simulink model "commhdlQPSKTxRxLoopback"  (R2025b)
settings: Solver=FixedStepDiscrete  StartTime=0.0  StopTime=0.03  RelTol=1e-3
PostLoadFcn:
  | hScopeConfig = get_param([gcs '/Receiver/QPSK Rx/Frequency and Time Synchronizer/Symbol Synchronizer/No HDL/QPSK Receiver Eye Diagram'],'ScopeConfiguration');
  | 
  | hScopeConfig.OpenAtSimulationStart = false;
  | hScopeConfig.Visible = false;
  | SamplesPerSymbol = 4;
  | %UpsamplesRx = 1;
  | clear hScopeConfig
InitFcn:
  | % RxAlign decoder latency (flat_simfix): 41 = netlist value used for HDL; set
  | % rxAlignLat = 25 in the base workspace before a model-level simulation.
  | if ~exist('rxAlignLat','var'), rxAlignLat = uint16(41); end
  | commhdlQPSKTxRxModelInit;
  | % Rate bridge: ADRV9002/Jupiter radio runs at 15.36 MHz = 2x the 7.68 MHz
  | % (4 samples/symbol @ Rsym=1.92 MHz) the QPSK Rx requires. The deployed
  | % Receiver must downsample the ADC stream by 2. UpsamplesRx=1 fed the QPSK
  | % Rx 8 sps (2x-upsampled) and broke symbol sync / the loopback bit check.
  | UpsamplesRx = 1;   %% T8 RATE FIX: rail 15.36e6 == ADC bus rate,
  | %% no ingress decimation (was 2 when the rail sat on the 7.68e6 rung)
  | UpsamplesTx = 1;
  | clear simTimingOffset;
StopFcn:
  | if exist('simTimingOffset','var')
  |   disp('Simulation completed');
  |   %QPSKTxRxVerification;
  | end
undefined symbols (not defined in the file or in its folder): Add, Config, fsym, randsrc, RandStream, Rsym, rxAlignLat, Shift
libraries: hdlsllib x141, simulink x45, dspsigops x30, dsphdlfiltering2 x6, dsphdlsigops2 x4, dsphdlmathfun2 x4, commdigbbndpm3 x4, dspmlti4 x2, commchan3 x1, commrflib2 x1, commcnvcod2 x1
(part 8 of 9)

== matlab function commhdlQPSKTxRxLoopback/TxRxComposite/Transmitter/Input Data/Message Generator/MATLAB Function ==
  data: enable input; reset input; out output; start output; stop output; valid output; count_out output; msg_count_out output
function [out, start, stop, valid, count_out, msg_count_out] = msggen(enable, reset)

persistent indexCount;
persistent toggle;
persistent msgCount;
persistent msgCountAll;
persistent msgCountBitIndex;

if isempty(indexCount) || isempty(toggle) || isempty(msgCount) || isempty(msgCountBitIndex) || isempty(msgCountAll)
    indexCount = uint32(0);
    msgCount = uint32(1);
    msgCountAll = uint32(1);
    msgCountBitIndex = uint8(0);
    toggle = false;
end

%% Constants -- FIXED pre-coded K=5 packet ROM (rom_words_1538_f3072.txt, 49216 bits,
%% word w = bits[32w..32w+31] MSB-first). Stored as 1538 x uint32 packed words
%% (a large inline logical literal crashes the Stateflow compiler),
%% unpacked into the 49216-element msgbits logical ROM and indexed with the
%% STOCK msgbits(indexCount+1) pattern. Replaces the stock 120-bit message ROM.
%% Content: K=5 [35 23] rate-1/2 coded info(24580)+tail(4) -> 49168 bits,
%% 3073x16 block-interleaved (perm r*16+c), + 48-bit PN9 filler. The K=5 Rx
%% deint(perm c*3073+r) + Viterbi(TB=25) recovers the 120-bit BIST message.
romWords = uint32([1204802801 1209539668 1975942268 2963809026 2596904318 4188557104 3596431864 4239974639 3463738471 2217388750 3654439215 3125256117 3023293192 2833794923 816778833 3181876726 1463245004 1536297995 531210280 521390638 503270692 25790812 3006566584 640748580 1552853862 3369715589 690379693 619729467 1586250071 2534918951 747314766 1864725699 736916321 2528559012 1966427766 2678711027 694905996 1090498697 4047016108 3888783770 1752854675 2327765102 4141019401 889360673 4078382531 606602352 3965635163 4041515764 2819874977 1574596945 321589146 384343845 752891311 2607187799 3958919490 4166073337 1201425593 865760697 4132523191 3234300202 319457634 4082652392 2743661104 3838643167 1212358201 3402087606 2198354590 3131288918 1003284279 1425529800 3391331687 3311587040 127937888 1089516081 3673635227 445764603 3537605218 797167348 4183576257 773960086 2766468030 4198128804 3458726264 2393905559 3489853414 2196393881 486375490 1145928153 3862936003 3396050587 2041684831 74224024 2508173738 3232951644 1850676608 575465608 2601014813 161140334 1224372193 2202544767 609459114 2299535289 1067761239 3728692708 1107255884 2941251540 3267112609 450986202 2552770051 2810502665 2112561500 1741574834 299210037 1512710571 2656835927 3574963367 4083599180 18682879 739084270 3764607777 1067439360 3750299744 515218676 2186757769 894832561 2742819396 1017874299 1616589898 3277014125 3903727308 3150698403 1763223118 1857536645 3533379933 3769362920 1004497246 1621852718 2953385647 670261293 650431976 3330551091 3243841717 2866634310 1783415789 2706704096 1229655886 1762424939 3329656707 692536697 2530874172 615889781 3641313861 3165276461 1575695498 1095991108 2393048602 2322677623 2462300094 672548471 443302646 2401744327 3195224733 2643525393 2032327687 4066687688 2052515282 525959574 1200737918 3120293673 2824716087 81481050 3706952732 3033304069 3294601023 1955426396 2406762541 3355246243 588796604 1217561840 532214079 2044577666 1032389574 1248771450 2328788581 791619531 3533714262 1280541402 1333456217 2856369162 2297528148 2544125963 2088596923 3884930713 1368671329 4087517486 159324756 651570540 2412111142 392114999 2370159585 908714534 2715295203 2682112071 2711284707 3728139541 2826127728 3139497352 3197213404 282717133 247483121 4130198852 3895374600 4237045182 424874395 3193515989 726780019 2770673358 3834366793 3393863207 1662254982 2163226171 1756225332 2918826582 1723191745 331423682 265369493 2248768111 193743543 1822232140 1188574963 2673534252 2654665973 33665318 2069877200 2095550304 687030672 3814367006 2518682845 2194284174 2210284937 2245819751 1262584459 280993686 3261008703 1628440877 915089377 3448523146 95732335 1313659002 1260523056 1000665243 2920058498 3059302077 4166433548 877848755 173376985 227198061 3363795968 1010180339 2461775866 3847670150 1698931964 2087397951 2527247761 425176101 3785411020 1349297358 2613815399 2392304903 3443745732 4261680018 2989926550 2661956505 833044881 3200424203 2681698098 1781916562 3524911335 3427913452 2480787959 3313609448 237605911 2668568412 4003366355 3127330044 1413351577 1831109279 846177568 4186381342 392587517 1317495262 1234132263 3207831315 2771924977 1663029718 3425889758 2739742993 1006198592 288020908 3490294386 3303183926 89484471 3533003533 335690994 902689980 3000871291 3889730770 3805817100 2857273051 63348295 572977109 1639313071 4158680949 1602817760 3709553447 3788468166 1773053108 1365908809 3700907952 1573591579 568463054 1879991147 69323806 440392871 2522583366 2710933589 150906642 3870974012 1886569819 2324535646 1507187207 2629501721 1760161311 35660463 2808287073 1143451145 2769391269 4173818791 1923310152 4232606257 669389120 1423207097 2046227766 3632023270 2198744970 3968414017 2395738869 1215433962 731322438 161964751 3293093619 224842784 3984933581 3121998056 2983752481 1433078765 2457641714 1631023948 1359402486 4227012072 4149592405 1687941922 2505970099 3983453067 307980754 2956380758 2117379389 2100280120 2035718660 258725890 4041819218 1949434289 175777631 2685890945 2936619036 1409909629 3043154311 2008052563 2411874163 2668314496 2611814908 3238904613 1657762836 2130246907 528734280 958809339 3836862512 8230316 1357805701 1477682684 1732389384 3117701793 3316638453 2358256083 2301059807 716088263 108771628 1140633043 1876044599 3771439014 787956565 1955170233 1754570785 1489848686 4019201518 2348900253 2081969428 3239156668 701792140 2894128036 1778726324 3538238998 1421524291 3537991122 1577794079 242894021 1356956559 1010995638 2442163953 2528844136 25202790 2486979355 662772831 822381038 1464695293 4294782743 3206584002 711024534 1324822961 2688654031 479697192 1169892583 2583377315 1635348899 157487841 3249790917 3502032110 410858799 335362838 3577961663 3223443922 3316423132 2283253993 2520994220 2885947309 3728000160 1695809603 1562878608 1301267166 2408164844 1302230188 3184675594 870494927 3904036614 3416157190 261484849 3964976954 2919737956 477639576 1420335417 1031608256 546934812 176155648 2873478944 2850789058 257123640 3640852739 3302294082 537046633 3129077721 1440937457 1649017228 3682906110 917465243 2621536216 3490813918 408762528 4277871199 303345609 3429261328 1781456717 994101137 3233202134 462971104 2186836563 3887379890 994553282 1519639102 1306273498 2107634001 1430641043 1248988685 2628225066 2546181794 2137684260 511177286 595738541 662776493 658185562 3369405162 529168517 2446864527 622256313 819681306 415328015 4113691780 534900412 2806458218 153784096 1202268017 3683991689 1377090874 3126297274 3545603267 1174213401 1463804439 216993290 1454157287 2826801417 2653565548 403961221 1654508340 954275206 1259686116 3453252826 3732323577 2410747618 2781486003 2858226441 1706504325 838562295 1184429697 314698179 1336032104 4276593890 1334804946 3876814892 2110413220 674760388 345149493 3378196395 4168579343 481251594 440319556 1607019172 3511452166 96512900 2896802245 3359778245 2653565757 535281887 648658714 1288320236 3646768756 60753304 2947838195 1459910118 3494212664 3725383650 1775233763 3715171596 3634419782 1864573308 1071068798 1334838154 4188248325 193444393 2339924786 4024130888 3662972727 968766718 959346415 4153644798 3639160359 3636849733 811995338 3131590300 2713579212 3303718022 3574250102 1396504649 1244044761 1378081383 812822708 542340745 538862408 3174610526 454115779 2989685913 2056749848 4104471819 760056897 3919070732 552523259 1071302743 2937668231 2282617100 4025888751 1976354404 2004033004 867727827 2155421527 1775607550 487082542 1069795780 2614602075 3484118902 335614148 2821194348 4072290021 1973749486 3369807218 1590065663 1514720505 1006765583 2049335206 1051783535 2968473493 684663495 3689960305 3333282694 4024463566 963991627 52211089 4119115897 3308432399 2469298186 3702609803 1463674664 3129611098 1475094431 380743536 4173335610 2923690251 4168372831 4074318299 3573722952 1227551570 1945617460 3188682481 1130457713 3836338573 2285857905 2662879320 3703031673 1843385953 3948298812 3432183889 835254942 930538225 4265504881 1307914106 345432724 1389149284 2498964923 200988725 4276973219 1835595416 1362825022 2577923270 238061094 1993869078 901341174 867489559 700052326 1333957091 4046510925 3532011587 536223879 1147407025 466374857 2847667437 2795823317 134613913 1972079339 125925492 81057330 2687942273 3093556331 4120910786 2485967932 2047140874 1041590264 2876183441 221213631 568597090 1212320458 4136460815 1248210961 2097701469 3768674233 2978685087 3617677831 2111207307 3745241564 1719042886 2152838467 269465709 3100095370 1596160290 3214601957 485882116 2561319758 2664762743 2766423900 3407324568 771934492 3728309352 1503163844 184762998 1496345397 2969468950 1727067881 622629482 167645933 325194033 74501931 205318352 1115326205 1124274385 1920293735 2001469635 445165137 3016544871 4248867883 3276869645 3313868698 3737138426 2063628009 4255733901 188155413 484702060 2848562425 4204433103 2278131640 3695057078 3375252164 1453715902 3786295219 2780461401 654125849 2626799110 3364787322 1390650888 1651817132 2081359570 1030002217 1246396635 1897703130 1542196505 646960413 3108998800 3267832361 147451240 1292168210 939441631 708260956 1068231395 2911330028 2783762739 2314125596 1533344163 4144296654 442759127 1884322937 1130924414 908315299 3261536962 2805752598 3321885594 3304687796 461645469 2658848112 3626039127 2461245286 763618243 3790393918 3066324139 3173713906 2992126282 1990724716 337986241 1789407253 22987792 4086127847 3228562568 3664457499 4261606902 2658157719 1777564265 4171671165 4175103858 2810529338 993856068 1459134663 1103703075 2411625273 575879518 2609343928 1972511260 345577472 2706576847 139974969 4118432466 3530027271 3853125088 3621809694 218725533 2988261449 871424681 222963540 2011072294 3733778211 2028568644 3118125258 3348863957 1318773733 1283462213 4293616597 1310709898 162769290 2501821043 1295831927 1498639911 2115883572 109431653 1497770867 20375250 1703289790 4195970274 899175526 2421894438 2816280534 3448527018 2173964134 2370841797 2405530599 1839799211 49806688 3951572939 3701379815 97727180 2522387928 3221018639 115760052 495216825 1471905024 1164712503 279065598 2486494152 3210631311 2541662795 3290956712 4173201560 2951442065 2398123248 2358968883 3680394943 273209594 1577699141 2110340655 2128338145 1767091768 4003213844 2674005339 2755971354 2759856494 777136466 2416529310 915198114 3918494261 179970576 3773434593 3490979523 819292424 4275310393 1714159194 3350498301 1562501207 422542082 947715171 2758251467 2324933845 4125369197 3123469432 2426592298 2680549074 1851281060 2248231552 146572812 900534439 2442015423 1362157204 3201817816 3366016907 4173839277 3785474750 2523229531 2390346862 510742672 1454910842 234900511 2031974073 338555629 4167251742 2903859384 2146554703 1919627351 998160787 1038327002 3797008050 1875176060 1166742039 2478398504 2592721825 886893418 2245589022 2056747411 207299859 4283369763 1748775293 1051096089 2585814632 2933423722 3469443613 20357305 3638937891 3623705238 258576962 1051752046 1582949444 1544361805 2343500339 3607688486 740604344 1235094596 2123776063 2184505536 856024743 2381424411 1141165357 3463739622 2741677513 1929714128 1319049685 2342472901 3880657182 3738880806 1545960332 2297891969 695249073 4097563110 3969693476 2365104016 850405100 2250147991 2937948299 628722389 2362945975 567819005 4087409965 2059072943 1393039718 3068729753 1087946277 990436966 3391255064 2309932146 3228006110 4128157119 1836661625 452696085 2708015652 2528088667 3239476764 1137624365 542654316 4269130292 3282568394 2631609029 3801472009 2859883842 3697213502 719108774 492314378 3543608234 620831893 1482939639 1222009594 3465267589 1864157100 1851902579 3091052741 785743232 995147633 3452252561 3294452505 2229861650 698045113 4222163023 2592937516 1718735990 242180948 2006408745 1412150379 3431652615 2662631667 3703654945 2010245237 1650234441 3102537096 2681591446 2312961596 1221718008 4201369170 4206775453 2441598447 832037648 2382650161 2791014231 2375135614 2948716823 2955585902 690979659 292513342 1157975458 2795219124 101302068 840768948 1414017486 407048397 21768117 3790149034 4272220897 2242099256 3338707065 1029041317 1789545807 3695127809 275769178 2520491969 1565610520 539169919 2153673086 3850539151 425556004 1755212310 1589159543 2267681895 3041870234 94786332 355023476 675822639 2437714269 988472681 4201766357 3226991306 3322005739 2911012271 1238751972 288277998 2507591037 1582493019 3847934904 486076937 567290429 3483638649 153855845 2496365353 3975299047 974638796 3998136232 989137960 1898917198 750196757 2586540626 934332385 1608094586 3290987748 1592334579 2841615470 1371570940 3364591972 2958416298 1918766067 931115645 3139101130 2241740414 2939234622 3477994516 2956068270 1714410721 1580873144 2901334196 3046220716 3642472080 1332650321 962896668 558744423 96158222 2299122273 1794634793 750168712 3610189895 3220794578 1915439211 1872017473 1509891327 3212468167 201806603 1975762227 4044408791 467175990 1526380547 297432424 3269881263 1305350767 3410823679 1598355310 1083799000 2333043718 2919619928 452310714 800829338 3977113668 3903703761 3562553559 3535807234 718603801 1792539630 3779294451 4031859642 840295908 2992725012 1488456151 4195414593 1727247261 273349209 1452262067 2228490773 3138650219 685103554 69832325 282401721 3754713272 858927835 1584900158 2801624880 1569742592 1457014287 3402815001 3239547415 4245140568 1669732407 715854453 3474520154 1906695421 4017347253 3209424503 1984886766 1506891898 156562404 1200393864 3061498374 1622813225 3713148192 146114142 973119239 3080063534 3945373241 3107663648 3267068684 3135414631 3282841547 2277571766 3568256230 1277495956 2721298484 1653390489 3968474135 1984340229 1156127326 2552269562 2223508240 1188823175 640740698 1274040201 2002844228 2441779658 703241295 4060571683 570670184 163243386 1260953124 974559708 3748149445 1835169943 1206653664 464491897 3390231634 3591647359 28813404 699894507 3688183141 4238050790 1374077723 990025906 3424668780 561113803 3304765826 1932625188 824889070 3515480717 1647026787 3748042851 926428395 2849622848 3441400675 2427762082 218304105 2783520378 3562996736 2650688348 143510873 638632259 2090196130 3396505857 1709408569 3262382177 634768598 952283853 1823489785 1071638287 10325130 150959118 310399008 2285140288 4227539673 2351514496 683780806 2901707019 1256072123 1643796108 251342443 2078744906 2566518341 1009582844 4139635136 3758144117 1784912520 2714112625 346921951 3482688842 844325715 1476729538 448590254 590847275 3810843062 1254731790 3597914101 2859906454 3081619232 1697441663 4273315064 3759554761 1279616305 1760931717 3182681103 1497890068 1411541561 1147583689 2696336651 2555260242 2873210750 952574294 968670822 4026216405 752839346 2167877236 911399443 2281316704 1829068740 1677018444 2144422183 1569841385 1485234138 3149247106 251070583 533609779 635472925 118607384 823507621 2871219985 3309591335 3937168287 381665869 2736872403 1312161062 218456103 986165389 3432660678 3916253777 1005375538 4071139872 2352715659 392826471 969442004 2918939281 1131322762 2119221688 1579542433 1947020568 2015783834 3334104598 3224492146 4183854482 1080417405 1036366614 612891250 3520546847 2123183290 1362947440 2074612778 2149876321 1109369504 1290823204 2676696245 1271392972 3670978798 3084932248 3842604037 2239132265 2623445850 2374943924 2420362389 1917524694 2509372725 2586972802 3646831646 4015459517 1453461158 1269968550 1577654521 1266920707 1237028445 2728581274 2949385620 3187737094 2736004866 234825071 2282991099 2248496021 3232522208 3019410794 2707311801 996007510 840101938 4254038590 3054561952 414681070 527840597 1728841015 4024925859 97933881 1445376372 1781335559 2892116704 3717628775 2194439858 970284772 1826419058 126008097 1380349619 2431993621 2287192630 2810130727 1211923045 1996581146 218181794 2115823121 1688536280 1724921507 1274841921 3016216633 2353005703 263102764 260979301 1262203912 3119892600 1705763523 1292853085 3010195100 415256652 2027469414 1163927630 4172521842 250219617 1392562676 836624874 1502799765 3736976180 3489286585 1384363470 2742176632 2909285275 4233011388 1341580250 2278477736 4249869053 1956200393 1742954963 339741992 847424959 2575336293 91484981 3526570439 3920494760 2717318180 4069529465 4105819601 2639573412 3711762896 2437335094 1449405311 500895507 2637802359 29389529 3764021124 3435708924 1775670478 2659558609 2995917878 742944662 3037676675 799088778 2533842456 1089420616 2463642138 1414515425 3155201593 992550426 2440737146 265398217 787265074 2540452797 2492023466 98151335 1875813918 4128480089 917500263 3892171995 2321740129 3470855003 1716980343 1560637483 1483790751 3125308144 3211266530 4274929516 297758672 1863773334 2587511598 2231279994 1453595773 1211550414 2374009761 980866375 3178830487 3343325167 3308206686 2879254869 1930247217 2194302351 667275304 570070688 3737681008 67595686 3689558531 2334311054 2581098046 4214813972 2443424592 1989197647 4287768507 452498210 4221667130 4039813738 3693432744 2890033887 1506755458 1478806147 1496737437 971085129 3383715523 2805855488 345336576 2971069199 1529843703 2490227837 705593196 3610973957 3173879169 1733510590 2504930362 1798940064 809349636 2943616113 3505641729 3655244539 2798312896 1994737988 2242114145 3197808889 2138384610 3126391676 3317929836 1165653316 3469544994 1930013970 3335817982 1244521841 938900329 2580660124 996687454 1902639454 1005591870 318256265 3765914446 2008582833 2012355776 3092211951 2255915317 201466349 3136420849 2774658193 2788317177 2908815235 3742839305]);
msgbitsLen = uint32(49216);   %% packed ROM: no unpacked bit array (Vivado 2025.1 crash at 49216 bits)

fullMessageLen = uint32(49216-1); %% Need the -1 to eat the feedback delay (stock hardcoded value in this model)

%% Logic
if enable && ~reset
    %% Set out data
    if indexCount < msgbitsLen %% Emit the fixed pre-coded packet bit (unpacked ROM)
        out = bitget(romWords(bitshift(indexCount, -5) + 1), 32 - bitand(indexCount, uint32(31))) ~= uint32(0);
        msgCountBitIndex = uint8(0);
    else %% beyond the ROM (should not occur: msgbitsLen==dataBitsPerPacket)
        out = false;
        msgCountBitIndex = uint8(0);
    end

    %% Flags
    start = indexCount == uint32(0);
    stop = indexCount == fullMessageLen;
    valid = true;

    %% Counters
    if fullMessageLen == indexCount
        if msgCount >= 9
            msgCount = uint32(1);
        else
            msgCount = msgCount +  1;
            msgCountAll = msgCountAll + 1;
        end
    end
    if indexCount <= fullMessageLen
        indexCount = indexCount + 1;
    end

else %% Enable == false

    if reset
        indexCount = uint32(0);
        msgCountBitIndex = uint8(0);
        toggle = false;
    end
    out = false;
    start = false;
    stop = false;
    valid = false;
end

if isempty(indexCount)
    count_out = uint32(0);
else
    count_out = indexCount;
end

msg_count_out = msgCountAll;

== matlab function commhdlQPSKTxRxLoopback/Receiver/QPSK Rx/Frequency and Time Synchronizer/Preamble Detector/FIFO/Validate Input Push Pop/MATLAB Function ==
  data: rst input; count output; enb input; dir input; initVal parameter; countToVal parameter
function count = hdlCounter(rst,enb,dir,initVal,countToVal)
%#codegen

persistent countReg

if(isempty(countReg))
    countReg = fi(initVal,0,nextpow2(countToVal+1),0);
end

if(rst)
    countReg(:) = initVal;
elseif(enb)
    if(dir)
        if(countReg==countToVal)
            countReg(:) = initVal;
        else
            countReg(:) = countReg+1;
        end
    else
        if(countReg==initVal)
            countReg(:) = countToVal;
        else
            countReg(:) = countReg-1;
        end
    end
end

count = countReg;

end

== matlab function commhdlQPSKTxRxLoopback/Receiver/QPSK Rx/Frequency and Time Synchronizer/Preamble Detector/FIFO/Validate Input Push Pop/No HDL/MATLAB Function ==
  data: pushFullDiag input; popEmptyDiag input; pushFull input; popEmpty input
function pushPopDiagnostics(pushFullDiag, popEmptyDiag, pushFull, popEmpty)
%#codegen


if(pushFull)
    switch pushFullDiag
        case 2
            warning('Push signal applied on full FIFO');
        case 3
            error('Push signal applied on full FIFO');
        otherwise
    end
end

if(popEmpty)
    switch popEmptyDiag
        case 2
            warning('Pop signal applied on empty FIFO');
        case 3
            error('Pop signal applied on empty FIFO');
        otherwise
    end
end

end

== matlab function commhdlQPSKTxRxLoopback/TxRxComposite/Transmitter/QPSK Tx/Bit Packetizer/Data Bits FIFO/MATLAB Function1 ==
  data: wr input; full output; rd input; dataBitsPerPacket parameter
function full = fcn(wr,rd,dataBitsPerPacket)
%#codegen
     
    depth = dataBitsPerPacket*2 - 1;
    persistent count;
    if isempty(count)
        count = fi(0,0,nextpow2(depth),0,hdlfimath);
    end

    % TXFIX_F3: saturating occupancy count.  The original wrapped at 65536 (and
    % underflowed at 0), which is how the fullRAM back-pressure runaway ends: the
    % producer keeps pushing until the uint16 count wraps and full drops again.
    % Simultaneous wr+rd stays a no-op, exactly as the original netted to.  131071
    % is the full range of count's fi(0,0,nextpow2(depth),0) = ufix17 type at this
    % rung (f1536: 65535 / the injector's 16'hFFFF); nextpow2 is NOT re-evaluated here.
    cntInc = wr;
    cntDec = rd;
    if cntInc && ~cntDec && (count ~= 131071)
        count(:) = count + 1;
    elseif cntDec && ~cntInc && (count ~= 0)
        count(:) = count - 1;
    end

    full = (count > depth);

end

== matlab function commhdlQPSKTxRxLoopback/Transmitter/QPSK Tx/Bit Packetizer/Data Bits FIFO/No HDL/MATLAB Function ==
  data: wr input; full output; rd input; ncount output; empty output; dataBitsPerPacket parameter
function [full,ncount,empty] = fcn(wr,rd,dataBitsPerPacket)
%#codegen
     
    depth = dataBitsPerPacket*2 - 1;
    persistent count;
    if isempty(count)
        count = fi(0,0,nextpow2(depth),0,hdlfimath);
    end

    empty = (count == 0);
    full = (count > depth);
    ncount = count;

    if wr
        count(:) = count + 1;
    end
    if rd
        count(:) = count - 1;
    end

end

== matlab function commhdlQPSKTxRxLoopback/TxRxComposite/Transmitter/QPSK Tx/Bit Packetizer/Data Bits FIFO/No HDL/MATLAB Function ==
  data: wr input; full output; rd input; ncount output; empty output; dataBitsPerPacket parameter
function [full,ncount,empty] = fcn(wr,rd,dataBitsPerPacket)
%#codegen
     
    depth = dataBitsPerPacket*2 - 1;
    persistent count;
    if isempty(count)
        count = fi(0,0,nextpow2(depth),0,hdlfimath);
    end

    empty = (count == 0);
    full = (count > depth);
    ncount = count;

    if wr
        count(:) = count + 1;
    end
    if rd
        count(:) = count - 1;
    end

end

== matlab function commhdlQPSKTxRxLoopback/TxRxComposite/Transmitter/QPSK Tx/Bit Packetizer/Data Bits FIFO/RAM Frame Status Indicator ==
  data: push input; out output; pop input; dataBitsPerPacket parameter
function out = fcn(push,pop,dataBitsPerPacket)

   persistent pushCount popCount frameCount;
   if isempty(pushCount)
       pushCount = fi(0,0,nextpow2(dataBitsPerPacket),0,hdlfimath);
       frameCount = fi(0,0,2,0,hdlfimath);
       popCount = fi(0,0,nextpow2(dataBitsPerPacket),0,hdlfimath);
   end
   
   % TXFIX_F2: saturating frameCount -- the original +1/-1 pair wrapped 3->0 on a
   % push-wrap and underflowed 0->3 on a pop-wrap.  A 3->0 wrap makes the pop-enable
   % latch read frameCount==0 and abort pops.  Simultaneous push-wrap and pop-wrap
   % stays a no-op, exactly as the original (+1 then -1) netted to.  3 is the full
   % range of frameCount's fi(0,0,2,0) type (the injector's 2'b11).
   fcInc = (pushCount == dataBitsPerPacket-1) && push;
   fcDec = (popCount == dataBitsPerPacket-1) && pop;
   if fcInc && ~fcDec && (frameCount ~= 3)
       frameCount(:) = frameCount + 1;
   elseif fcDec && ~fcInc && (frameCount ~= 0)
       frameCount(:) = frameCount - 1;
   end

   if push
       if pushCount == dataBitsPerPacket - 1
           pushCount(:) = 0;
       else
           pushCount(:) = pushCount + 1;
       end
   end

   if pop 
       if popCount == dataBitsPerPacket - 1
           popCount(:) = 0;
       else
           popCount(:) = popCount + 1;
       end
   end

   out = frameCount;

end

== matlab function commhdlQPSKTxRxLoopback/TxRxComposite/Receiver/Capture Data Bits/MATLAB Function ==
  data: valid input; datain input; start input; stop input; count_out output; packets_out output; bit_errors_out output
function [count_out, packets_out, bit_errors_out] = msgdec(valid, datain, start, stop)

persistent count;
persistent msgbuffer;

persistent packetsReceived
persistent errors;

if isempty(count) || isempty(msgbuffer) || isempty(packetsReceived)
    count = uint32(0);
    msgbuffer = zeros(1,120+8)>0; % ADI Hello WorldX
    packetsReceived = uint32(0);
    errors = uint32(0);
end

% Mesg
strAscii = dec2bin('ADI Hello World',8);
msgarray = reshape(strAscii', [1, numel(strAscii)]);
msgbits = logical(msgarray - 48);

% msgLen = uint32(2240);

if valid
    if start
        count = uint32(1);
        packetsReceived = packetsReceived + 1;
    end

    if count <= (length(msgbuffer) - 8)
        msgbuffer(count) = datain;
        if datain ~= msgbits(count)
            errors = errors + 1;
        end

    elseif count == length(msgbuffer) + 1
    end
    
    if count <= length(msgbuffer) + 2
        count = count + 1;
    end
end

count_out = count;
packets_out = packetsReceived;
bit_errors_out = errors;

== matlab function commhdlQPSKTxRxLoopback/TxRxComposite/Receiver/QPSK Rx/Frequency and Time Synchronizer/Packet Controller/MATLAB Function ==
  data: valid input; syncPulse input; out output
function out = fcn(valid,syncPulse)
%#codegen

  persistent Reg;
  if isempty(Reg)
      Reg = false;
  end
  
  out = Reg;
  
  if Reg && valid
      Reg = false;
  end
  
  if syncPulse
      Reg = true;
  end
  
end

== matlab function commhdlQPSKTxRxLoopback/TxRxComposite/Receiver/QPSK Rx/Frequency and Time Synchronizer/Packet Controller/sample discard controller ==
  data: dataIn input; validIn input; dataOut output; startIn input; endIn input; startOut output; endOut output; validOut output
function [dataOut,startOut,endOut,validOut] = controller(dataIn,validIn,startIn,endIn)
%#codegen

   persistent active dataOutReg validOutReg startOutReg endOutReg;
   if isempty(active)
      active  = false;
      dataOutReg = cast(0,'like',dataIn);
      validOutReg = false;
      startOutReg = false;
      endOutReg = false;
   end
   
   dataOut = dataOutReg;
   validOut = validOutReg;
   startOut = startOutReg;
   endOut = endOutReg;
   
   startOutReg = startIn;
   endOutReg = endIn;
   
   if startIn
       active = true;
   end
   
   if active
       dataOutReg(:) = dataIn;
       validOutReg = validIn;
   else
       dataOutReg(:) = 0;
       validOutReg = false;
   end
   
   if endIn
       if active 
           endOutReg = true;
       else
           endOutReg = false;
       end
       active = false;
   end
end

== matlab function commhdlQPSKTxRxLoopback/TxRxComposite/Receiver/QPSK Rx/Frequency and Time Synchronizer/Preamble Detector/Correlator/ThresholdLimiter ==
  settings: fimath=hdlfimath
  data: x input; y output
function y = applyLowerLimit(x)
    % Apply a lower limit to the threshold.
    %#codegen
    
    % Threshold is computed by summing across 63 samples.
    % Set lower limit to be equivalent of all 63 samples
    % having their LSB set to 1 and all others set to 0. 
    lowerLimit = cast(0.01, 'like', x);
    
    if x < lowerLimit
        y = lowerLimit;
    else
        y = x;
    end
end

== matlab function commhdlQPSKTxRxLoopback/TxRxComposite/Receiver/QPSK Rx/Frequency and Time Synchronizer/Preamble Detector/FIFO/Validate Input Push Pop/MATLAB Function ==
  data: rst input; count output; enb input; dir input; initVal parameter; countToVal parameter
function count = hdlCounter(rst,enb,dir,initVal,countToVal)
%#codegen

persistent countReg

if(isempty(countReg))
    countReg = fi(initVal,0,nextpow2(countToVal+1),0);
end

if(rst)
    countReg(:) = initVal;
elseif(enb)
    if(dir)
        if(countReg==countToVal)
            countReg(:) = initVal;
        else
            countReg(:) = countReg+1;
        end
    else
        if(countReg==initVal)
            countReg(:) = countToVal;
        else
            countReg(:) = countReg-1;
        end
    end
end

count = countReg;

end

== matlab function commhdlQPSKTxRxLoopback/TxRxComposite/Receiver/QPSK Rx/Frequency and Time Synchronizer/Preamble Detector/FIFO/Validate Input Push Pop/No HDL/MATLAB Function ==
  data: pushFullDiag input; popEmptyDiag input; pushFull input; popEmpty input
function pushPopDiagnostics(pushFullDiag, popEmptyDiag, pushFull, popEmpty)
%#codegen


if(pushFull)
    switch pushFullDiag
        case 2
            warning('Push signal applied on full FIFO');
        case 3
            error('Push signal applied on full FIFO');
        otherwise
    end
end

if(popEmpty)
    switch popEmptyDiag
        case 2
            warning('Pop signal applied on empty FIFO');
        case 3
            error('Pop signal applied on empty FIFO');
        otherwise
    end
end

end

== matlab function commhdlQPSKTxRxLoopback/Receiver/QPSK Rx/Frequency and Time Synchronizer/Packet Controller/MATLAB Function ==
  data: valid input; syncPulse input; out output
function out = fcn(valid,syncPulse)
%#codegen

  persistent Reg;
  if isempty(Reg)
      Reg = false;
  end
  
  out = Reg;
  
  if Reg && valid
      Reg = false;
  end
  
  if syncPulse
      Reg = true;
  end
  
end

== matlab function commhdlQPSKTxRxLoopback/TxRxComposite/Receiver/QPSK Rx/Frequency and Time Synchronizer/Symbol Synchronizer/Interpolation Control ==
  data: mu output; Delta input; Underflow output
function [mu,Underflow] = Interpolation_ctrl(Delta)
% Implementation of modulo-1 counter for interpolation control listed in
% Figure 8.4.19 of "Digital Communications - A Discrete-Time Approach"
% by Michael Rice. See design details in Chapter 8.4.3 of the same book.
% 
% Input:
%   Delta - Loop filter output. If loop is in lock, delta would be small
% Output:
%   Underflow - Indicator of counter underflow. This is the strobe signal
%               for downstream processing
%   mu - Difference between actual sampling instant and the optimal instant,
%        between zero and one
%#codegen

% countReg - Counter value delayed by 1 sample
% muReg - The estimated timing error normalized by half QPSK symbols

   mask = fi(1-2^(-10),1,11,10);
   
   persistent countReg underflowReg muReg;
   if isempty(countReg)
       countReg  = fi(0,1,11,10);
       muReg = fi(0,1,11,10);
       underflowReg = false;
   end
   
   
   Underflow = underflowReg;
   mu = muReg;   
   
   
      % T8.4 anti-wedge clamp: if Delta <= -0.125 the decrementing counter
   % never underflows (strobes stop FOREVER -- Class-4 wedge / Class-1
   % episode mechanism; see tb_timing_wedge.v). Bound Delta so the
   % counter always decrements by >= 1 LSB.
   wlim = fi(511/1024,1,11,10);
   if Delta > wlim
       Delta = wlim;
   elseif Delta < -wlim
       Delta = fi(-511/1024,1,11,10);
   end
   counter = bitand(mask,countReg)-Delta-fi(0.5,1,11,10); % decrementing counter
   
   % if countReg is a nonnegative number,
   % then mod(countReg,1) equals the fractional part of countReg
   if counter < 0
       underflowReg = true;
       muReg = bitshift(bitand(mask,countReg),1);
       countReg = fi(counter+1,1,11,10);% create underflow to counter
   else
       underflowReg = false;
       countReg = fi(counter,1,11,10);
   end
   


end

== matlab function commhdlQPSKTxRxLoopback/TxRxComposite/Receiver/QPSK Rx/Frequency and Time Synchronizer/Symbol Synchronizer/Rate Handle/FIFO/Validate Input Push Pop/MATLAB Function ==
  data: rst input; count output; enb input; dir input; initVal parameter; countToVal parameter
function count = hdlCounter(rst,enb,dir,initVal,countToVal)
%#codegen

persistent countReg

if(isempty(countReg))
    countReg = fi(initVal,0,nextpow2(countToVal+1),0);
end

if(rst)
    countReg(:) = initVal;
elseif(enb)
    if(dir)
        if(countReg==countToVal)
            countReg(:) = initVal;
        else
            countReg(:) = countReg+1;
        end
    else
        if(countReg==initVal)
            countReg(:) = countToVal;
        else
            countReg(:) = countReg-1;
        end
    end
end

count = countReg;

end

== matlab function commhdlQPSKTxRxLoopback/TxRxComposite/Receiver/QPSK Rx/Frequency and Time Synchronizer/Symbol Synchronizer/Rate Handle/FIFO/Validate Input Push Pop/No HDL/MATLAB Function ==
  data: pushFullDiag input; popEmptyDiag input; pushFull input; popEmpty input
function pushPopDiagnostics(pushFullDiag, popEmptyDiag, pushFull, popEmpty)
%#codegen


if(pushFull)
    switch pushFullDiag
        case 2
            warning('Push signal applied on full FIFO');
        case 3
            error('Push signal applied on full FIFO');
        otherwise
    end
end

if(popEmpty)
    switch popEmptyDiag
        case 2
            warning('Pop signal applied on empty FIFO');
        case 3
            error('Pop signal applied on empty FIFO');
        otherwise
    end
end

end

== matlab function commhdlQPSKTxRxLoopback/TxRxComposite/Receiver/QPSK Rx/FEC Decoder Wrapper/RxDeint ==
  data: dataIn input; codedPair output; startIn input; endIn input; validIn input; vitReset output; deintValid output; frameStart output; frameEnd output
function [codedPair, vitReset, deintValid, frameStart, frameEnd] = fecRxDeint(dataIn, startIn, endIn, validIn)
%#codegen
persistent ramA ramB rdBank wptr pcnt hold0 hold1 rdGate rcol rrow;
CODED=uint16(49168); COLS=uint16(16); ROWS=uint16(3073);
NPAIR=uint16(24584);
if isempty(ramA), ramA=fi(zeros(1,49168),0,1,0); ramB=fi(zeros(1,49168),0,1,0); rdBank=false; wptr=uint16(0); pcnt=uint16(0); hold0=fi(0,0,1,0); hold1=fi(0,0,1,0); rdGate=false; rcol=uint16(0); rrow=uint16(0); end
rb=rdBank; w=wptr; pc=pcnt; g=rdGate; h0=hold0; h1=hold1; cc=rcol; rr=rrow;
pair0=h0; pair1=h1;
vitReset=false; deintValid=false; frameStart=false; frameEnd=false;
wrPos=uint16(65535); wrBit=fi(0,0,1,0); wrBankA=false; doWr=false;
if validIn
  if startIn, w=uint16(0); pc=uint16(0); rb=~rb; g=true; cc=uint16(0); rr=uint16(0); end % rdGate=TRUE: frame pair0 read COINCIDES with frameStart (RxAlign arms on that beat); read-counters reset in lockstep with pc
  % ---- READ side first (opposite bank; RXROOT E8 isolated reads: 1 pair per 2 validIn beats) ----
  if g && (pc < NPAIR)
    % divisionless read address: cc (even col) / rr (row) are incremental counters.
    % rc0=2*pc is even so rc1=rc0+1 keeps the same row -> perm1 = perm0 + ROWS (one add).
    perm0 = cc*ROWS + rr;
    perm1 = perm0 + ROWS;
    b0v = fi(0,0,1,0); b1v = fi(0,0,1,0);
    if perm0 < CODED
      if rb, b0v = ramB(double(perm0)+1); else b0v = ramA(double(perm0)+1); end
    end
    if perm1 < CODED
      if rb, b1v = ramB(double(perm1)+1); else b1v = ramA(double(perm1)+1); end
    end
    pair0 = b0v; pair1 = b1v; h0 = b0v; h1 = b1v;
    deintValid = true;
    if pc == uint16(0), vitReset = true; end
    pc = pc + 1;
    cc = cc + uint16(2);
    if cc == COLS, cc = uint16(0); rr = rr + uint16(1); end
  end
  % ---- WRITE side after all reads ----
  if w < CODED
    wrPos = w; wrBit = fi(dataIn,0,1,0); wrBankA = rb; doWr = true;
    w = w + 1;
  end
  g = ~g;
  frameStart=startIn; frameEnd=endIn;
end
codedPair = fi([pair0; pair1], 0, 1, 0);
% ---- persist state last ----
if doWr
  if wrBankA, ramA(double(wrPos)+1)=wrBit; else ramB(double(wrPos)+1)=wrBit; end
end
rdBank=rb; wptr=w; pcnt=pc; rdGate=g; hold0=h0; hold1=h1; rcol=cc; rrow=rr;

== matlab function commhdlQPSKTxRxLoopback/TxRxComposite/Receiver/QPSK Rx/FEC Decoder Wrapper/RxAlign ==
  data: decBit input; dataOut output; deintValid input; frameStart input; frameEnd input; skipCount input; startOut output; endOut output; validOut output; alignLat input
function [dataOut, startOut, endOut, validOut] = fecRxAlign(decBit, deintValid, frameStart, frameEnd, skipCount, alignLat)
%#codegen
persistent oc started skip;
INFO=uint16(24580);
if isempty(oc), oc=uint16(0); started=false; skip=uint16(0); end
o=oc; st=started; sk=skip;
dataOut=false; startOut=false; endOut=false; validOut=false;
sc = uint16(skipCount);
if sc > INFO, sc = INFO; end
if deintValid
  if frameStart, o=uint16(0); st=true; sk=sc+uint16(alignLat); end % alignLat = gated-Viterbi latency in deintValid beats incl. VitGate hold reg (RXROOT E8): 41 on the netlist, 25 for the behavioural Viterbi in model sim (rxAlignLat)
  if st
    if sk > uint16(0)
      sk = sk - uint16(1);
    elseif o < INFO
      dataOut = decBit;
      startOut = (o==uint16(0));
      endOut   = (o==(INFO-1));
      validOut = true;
      o = o + uint16(1);
    end
  end
end
oc=o; started=st; skip=sk;

== matlab function commhdlQPSKTxRxLoopback/TxRxComposite/Receiver/QPSK Rx/FEC Decoder Wrapper/FecCounters ==
  data: e1 input; c1 output; e2 input; e3 input; e4 input; e5 input; e6 input; c2 output; c3 output; c4 output; c5 output; c6 output
function [c1, c2, c3, c4, c5, c6] = fecCounters(e1, e2, e3, e4, e5, e6)
%#codegen
% Free-running FEC-Rx datapath event counters (reset by modem soft-reset 0x000).
persistent k1 k2 k3 k4 k5 k6;
if isempty(k1)
  k1=uint32(0); k2=uint32(0); k3=uint32(0); k4=uint32(0); k5=uint32(0); k6=uint32(0);
end
MAX=uint32(4294967295);
n1=k1; n2=k2; n3=k3; n4=k4; n5=k5; n6=k6;
if e1 && n1<MAX, n1=n1+uint32(1); end
if e2 && n2<MAX, n2=n2+uint32(1); end
if e3 && n3<MAX, n3=n3+uint32(1); end
if e4 && n4<MAX, n4=n4+uint32(1); end
if e5 && n5<MAX, n5=n5+uint32(1); end
if e6 && n6<MAX, n6=n6+uint32(1); end
c1=n1; c2=n2; c3=n3; c4=n4; c5=n5; c6=n6;
k1=n1; k2=n2; k3=n3; k4=n4; k5=n5; k6=n6;

== matlab function commhdlQPSKTxRxLoopback/Receiver/QPSK Rx/Frequency and Time Synchronizer/Symbol Synchronizer/Rate Handle/FIFO/Validate Input Push Pop/MATLAB Function ==
  data: rst input; count output; enb input; dir input; initVal parameter; countToVal parameter
function count = hdlCounter(rst,enb,dir,initVal,countToVal)
%#codegen

persistent countReg

if(isempty(countReg))
    countReg = fi(initVal,0,nextpow2(countToVal+1),0);
end

if(rst)
    countReg(:) = initVal;
elseif(enb)
    if(dir)
        if(countReg==countToVal)
            countReg(:) = initVal;
        else
            countReg(:) = countReg+1;
        end
    else
        if(countReg==initVal)
            countReg(:) = countToVal;
        else
            countReg(:) = countReg-1;
        end
    end
end

count = countReg;

end

== matlab function commhdlQPSKTxRxLoopback/TxRxComposite/Receiver/QPSK Rx/FEC Decoder Wrapper/FecCapture ==
  data: bitsIn input; capIn output; validIn input; startIn input; codedPair input; deintValid input; decBit input; skipCount input; outValid input; capDeint output; capOut output
function [capIn, capDeint, capOut] = fecCapture(bitsIn, validIn, startIn, codedPair, deintValid, decBit, skipCount, outValid)
%#codegen
persistent rIn rDe rOu nIn nDe nOu armIn skp;
if isempty(rIn)
  rIn=uint32(0); rDe=uint32(0); rOu=uint32(0);
  nIn=uint16(0); nDe=uint16(0); nOu=uint16(0); armIn=false; skp=uint16(0);
end
% sync-semantics compliant (RXROOT E11c): locals, persist last.
a=rIn; b=rDe; c=rOu; xIn=nIn; xDe=nDe; xOu=nOu; arm=armIn; sk=skp; %#ok<NASGU>
% --- CAP_IN: first 32 coded-in bits, armed at startIn, gated by validIn ---
if validIn
  if startIn, xIn=uint16(0); a=uint32(0); arm=true; end
  if arm && xIn < uint16(32)
    if bitsIn, a = bitor(a, bitshift(uint32(1), double(xIn))); end
    xIn = xIn + uint16(1);
  end
end
% --- CAP_DEINT: first 32 deint-output coded bits (2 per pair), gated by deintValid ---
if startIn, xDe=uint16(0); b=uint32(0); end
if deintValid && xDe < uint16(32)
  b0 = codedPair(1) ~= 0; b1 = codedPair(2) ~= 0;
  if b0, b = bitor(b, bitshift(uint32(1), double(xDe))); end
  xDe = xDe + uint16(1);
  if xDe < uint16(32)
    if b1, b = bitor(b, bitshift(uint32(1), double(xDe))); end
    xDe = xDe + uint16(1);
  end
end
% --- CAP_OUT (RXROOT E8): first 32 bits of the WRAPPER OUTPUT stream ---
% i6 = RxAlign dataOut gated by i8 = RxAlign validOut: exactly the bits the
% BIST compares, alignment-independent. Golden expectation 0x04922282.
sc = uint16(skipCount); sk = uint16(0); %#ok<NASGU>
if startIn, xOu=uint16(0); c=uint32(0); end
if outValid && xOu < uint16(32)
  if decBit, c = bitor(c, bitshift(uint32(1), double(xOu))); end
  xOu = xOu + uint16(1);
end
capIn = a; capDeint = b; capOut = c;
rIn=a; rDe=b; rOu=c; nIn=xIn; nDe=xDe; nOu=xOu; armIn=arm; skp=sk;

== matlab function commhdlQPSKTxRxLoopback/TxRxComposite/Receiver/QPSK Rx/FecCaptureCadence ==
  data: startIn input; capCad output; validIn input
function capCad = fecCaptureCadence(startIn, validIn)
%#codegen
persistent sCnt gap snv vrun seenStart sawValid measuring;
if isempty(sCnt)
  sCnt=uint8(0); gap=uint8(0); snv=uint8(0); vrun=uint8(0);
  seenStart=false; sawValid=false; measuring=false;
end
% sync-semantics compliant (RXROOT E11c): locals, persist last.
sC=sCnt; gp=gap; sv=snv; vr=vrun; seen=seenStart; saw=sawValid; mea=measuring;
if startIn
  if sC < uint8(255), sC = sC + uint8(1); end
  if ~validIn && sv < uint8(255), sv = sv + uint8(1); end
  if ~seen
    seen = true; mea = true; gp = uint8(0); saw=false; vr=uint8(0);
  end
end
if mea && ~saw
  if validIn
    saw = true;
  elseif gp < uint8(255)
    gp = gp + uint8(1);
  end
end
if seen && validIn && vr < uint8(255)
  vr = vr + uint8(1);
end
capCad = bitor(bitor(uint32(sC), bitshift(uint32(gp),8)), bitor(bitshift(uint32(sv),16), bitshift(uint32(vr),24)));
sCnt=sC; gap=gp; snv=sv; vrun=vr; seenStart=seen; sawValid=saw; measuring=mea;

== matlab function commhdlQPSKTxRxLoopback/TxRxComposite/Receiver/QPSK Rx/RstCsCounter ==
  data: e input; c output
function c = rstCsCount(e)
%#codegen
% Count RISING EDGES of the CFO-step-detector carrier-sync reset (AXI 0x150).
% Saturating; reset by the modem soft-reset 0x000 via the persistent init.
persistent prev cnt;
if isempty(prev), prev = false; cnt = uint32(0); end
n = cnt;
if e && ~prev && n < uint32(4294967295)
    n = n + uint32(1);
end
c = n;
cnt = n;
prev = logical(e);

== matlab function commhdlQPSKTxRxLoopback/TxRxComposite/Transmitter/Input Data/ByteBitShifter ==
  data: enable input; bit output; reset input; start input; extWord input; extWordAvail input; extWordFirst input; popToggle output; txur output
function [bit, popToggle, txur] = byteBitShifterBlk(enable, reset, start, extWord, extWordAvail, extWordFirst)
% Block wrapper around qpskByteBitShifterStrict (the unit-tested single source
% of truth). Persistent state only; the effective enable matches the
% Message Generator chart's active condition (enable && ~reset) so the
% shifter emits bits on exactly the generator's bit steps. pop is
% exported as a toggle (one flip per word latch OR discard) to survive
% the slow->fast rate crossing; upstream edge-detects it into a pulse.
% txur (framestat TX-underrun witness): one-step pulse when the shifter
% hit its UNDERFLOW reload -- the only aligned->unaligned transition
% without a pop (the strict phase-error discard pops). Zeros air.
persistent state tog
if isempty(state)
    state = qpskByteBitShifterStrict();
    tog = false;
end
en = logical(enable) && ~logical(reset);
wasAligned = state.aligned;
[bit, pop, state] = qpskByteBitShifterStrict(state, en, logical(start), ...
    uint64(extWord), logical(extWordAvail), logical(extWordFirst), true);
if pop
    tog = ~tog;
end
popToggle = tog;
txur = wasAligned && ~state.aligned && ~pop;

== matlab function commhdlQPSKTxRxLoopback/TxRxComposite/Transmitter/Input Data/FEC Tx Encoder K5/TxGateK5 ==
  data: bitIn input; infoBit output; enable input; reset input; start input; encReset output; infoValid output; beatIdx output; frameValid output; frameStart output
function [infoBit, encReset, infoValid, beatIdx, frameValid, frameStart] = fecTxGateK5(bitIn, enable, reset, start)
%#codegen
% sync-semantics (RXROOT E11c): locals in, outputs from locals, persist last.
persistent beat armed;
INFO=uint16(24580); NIN=uint16(24584); PAYLOAD=uint16(49216);
if isempty(beat), beat=uint16(0); armed=false; end
b=beat; a=armed;
infoBit=false; encReset=false; infoValid=false; beatIdx=uint16(0);
frameValid=false; frameStart=false;
en = logical(enable) && ~logical(reset);
if en
  if start, b=uint16(0); a=true; encReset=true; end
  if a
    if b < INFO
      infoBit = logical(bitIn); infoValid = true;
    elseif b < NIN
      infoBit = false;          infoValid = true;   % K-1 zero tail flush
    end
    beatIdx = b; frameValid = true; frameStart = (b==uint16(0));
    if b < PAYLOAD-uint16(1), b=b+uint16(1); else, b=uint16(0); end
  end
end
beat=b; armed=a;

== matlab function commhdlQPSKTxRxLoopback/TxRxComposite/Transmitter/Input Data/FEC Tx Encoder K5/ConvEncK5 ==
  data: infoBit input; codedPair output; encReset input; infoValid input
function codedPair = fecConvEncK5(infoBit, encReset, infoValid)
%#codegen
persistent sr;
if isempty(sr), sr = false(1,4); end
srUse = sr;
if encReset, srUse = false(1,4); end   % reset-then-advance (zero frame state)
in = logical(infoBit);
s0=in; s1=srUse(1); s2=srUse(2); s3=srUse(3); s4=srUse(4);
g0 = xor(s0, xor(s1, xor(s2, s4)));   % poly 35 oct = 11101
g1 = xor(s0, xor(s3, s4));            % poly 23 oct = 10011
codedPair = [g0; g1];
% state update: advance ONLY on infoValid, else HOLD (anti-zero-stuff gate)
if infoValid
  sr = [in, srUse(1:3)];
else
  sr = srUse;
end
